simulink library "sm_car_scene_slalom"  (R2026a)
settings: Solver=VariableStepAuto
undefined symbols (not defined in the file or in its folder): Maneuver, Scene, X, Y, Z
libraries: sm_lib x4, Scene_Utilities x3
Description:
  | Scene of Simscape Vehicle Templates Library
  | 
  | Copyright 2018-2026 The MathWorks, Inc.
settings Model: Creator=smiller  LastModifiedBy=smiller

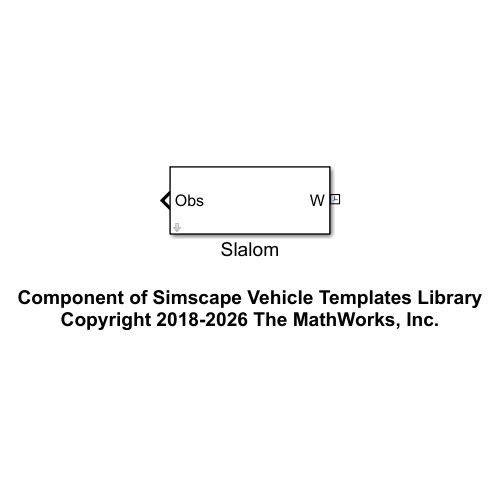
[thumbnail: Simulink's stored preview of the top-level diagram]
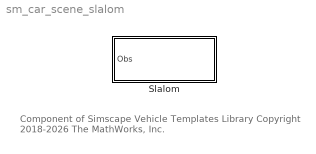
== system sm_car_scene_slalom ==
  note: Component of Simscape Vehicle Templates Library
      | Copyright 2018-2026 The MathWorks, Inc.
  Slalom : Subsystem  mask(Slalom Course){road=Scene.Slalom.Road, dashes=Scene.Slalom.Dashes, cones=Scene.Slalom.Cones, vehTraj=Maneuver.Trajectory}
      mask prompts: road "Road (structure)"; dashes "Dashes (structure)"; cones "Cones (structure)"; vehTraj "Path (structure)"
      mask help: Series of cones in a straight line intended for a slalom maneuver.

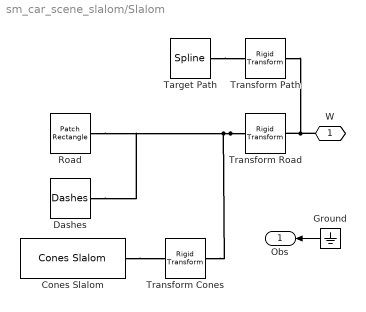
== system sm_car_scene_slalom/Slalom ==
  Cones Slalom : Scene_Utilities/Cones Slalom  y_cones=cones.Placement.xLatOffset.Value  x_cone_1=cones.Placement.xCone1.Value  x_cone_spacing=cones.Placement.xSpacing.Value  num_cones=cones.Placement.nCones.Value  height=0.6  baseThickness=0.04  baseWidth=0.5  coneBaseDiameter=0.24  coneTopDiameter=0.06  reflectiveStripHeight=0.3  coneColor=[248 78 25]/255  reflectiveStripColor=[0.75 0.75 0.75]
  Dashes : Scene_Utilities/Dashes  dash_pitch=dashes.pitch  num_dashes=dashes.num  dash_l=dashes.l  dash_h=dashes.h  dash_w=dashes.w  thickness_base=dashes.base_h  dash_clr=dashes.clr  dash_opc=dashes.opc
  Ground : Ground
  Road : Scene_Utilities/Patch Rectangle  gp_l=road.l  gp_w=road.w  gp_h=road.h  gp_clr=road.clr  gp_opc=road.opc
  Target Path : sm_lib/Curves and Surfaces/Spline  DataPoints=[vehTraj.x.Value' vehTraj.y.Value' vehTraj.z.Value']  DataPointsUnits=m  EndConditionType=Natural  GraphicType=FromGeometry  MarkerShape=Sphere  MarkerSize=10  GraphicVisPropType=SimpleVisualProperties  GraphicDiffuseColor=[0.0 0.0 0.0]  GraphicOpacity=1.0  GraphicSpecularColor=[0.5 0.5 0.5 1.0]  GraphicAmbientColor=[0.15 0.15 0.15 1.0]  GraphicEmissiveColor=[0.0 0.0 0.0 1.0]  GraphicShininess=75
  Transform Cones : sm_lib/Frames and Transforms/Rigid Transform  RotationMethod=None  FollAlignAxisA=+X  BaseAlignAxisA=+Y  FollAlignAxisB=+Y  BaseAlignAxisB=+Z  RotationStandardAxis=+Z  RotationAngle=0.0  RotationAngleUnits=deg  RotationArbitraryAxis=[0 0 1]  RotationSequenceAxes=FollowerAxes  RotationSequence=XYX  RotationSequenceAngles=[0 0 0]  RotationSequenceAnglesUnits=deg  RotationMatrix=[1 0 0; 0 1 0; 0 0 1]  Quaternion=[1 0 0 0]  TranslationMethod=StandardAxis  TranslationCartesianOffset=[0 0 0]  TranslationCartesianOffsetUnits=m  TranslationStandardAxis=-X  TranslationStandardOffset=road.x  TranslationStandardOffsetUnits=m  TranslationROffset=0  TranslationROffsetUnits=m  TranslationThetaOffset=0  TranslationThetaOffsetUnits=deg  TranslationZOffset=0  TranslationZOffsetUnits=m
  Transform Path : sm_lib/Frames and Transforms/Rigid Transform  RotationMethod=None  FollAlignAxisA=+X  BaseAlignAxisA=+Y  FollAlignAxisB=+Y  BaseAlignAxisB=+Z  RotationStandardAxis=+Z  RotationAngle=0.0  RotationAngleUnits=deg  RotationArbitraryAxis=[0 0 1]  RotationSequenceAxes=FollowerAxes  RotationSequence=XYX  RotationSequenceAngles=[0 0 0]  RotationSequenceAnglesUnits=deg  RotationMatrix=[1 0 0; 0 1 0; 0 0 1]  Quaternion=[1 0 0 0]  TranslationMethod=StandardAxis  TranslationCartesianOffset=[0 0 0]  TranslationCartesianOffsetUnits=m  TranslationStandardAxis=+Z  TranslationStandardOffset=road.h  TranslationStandardOffsetUnits=m  TranslationROffset=0  TranslationROffsetUnits=m  TranslationThetaOffset=0  TranslationThetaOffsetUnits=deg  TranslationZOffset=0  TranslationZOffsetUnits=m
  Transform Road : sm_lib/Frames and Transforms/Rigid Transform  RotationMethod=RotationSequence  FollAlignAxisA=+X  BaseAlignAxisA=+Y  FollAlignAxisB=+Y  BaseAlignAxisB=+Z  RotationStandardAxis=+Z  RotationAngle=0.0  RotationAngleUnits=deg  RotationArbitraryAxis=[0 0 1]  RotationSequenceAxes=BaseAxes  RotationSequence=ZYX  RotationSequenceAngles=[road.yaw road.pitch road.roll]  RotationSequenceAnglesUnits=rad  RotationMatrix=[1 0 0; 0 1 0; 0 0 1]  Quaternion=[1 0 0 0]  TranslationMethod=Cartesian  TranslationCartesianOffset=[road.x road.y road.z]  TranslationCartesianOffsetUnits=m  TranslationStandardAxis=+Z  TranslationStandardOffset=0  TranslationStandardOffsetUnits=m  TranslationROffset=0  TranslationROffsetUnits=m  TranslationThetaOffset=0  TranslationThetaOffsetUnits=deg  TranslationZOffset=0  TranslationZOffsetUnits=m
  W : PMIOPort  Side=Left
  Obs : Outport  VectorParamsAs1DForOutWhenUnconnected=off
  wires:
  Ground/1 -> Obs/1
  connections:
  Cones Slalom/LConn1 -- Transform Cones/RConn1
  Transform Road/RConn1 -- Transform Cones/LConn1 -- Road/RConn1 -- Dashes/LConn1
  W/RConn1 -- Transform Path/LConn1 -- Transform Road/LConn1
  Target Path/LConn1 -- Transform Path/RConn1
